simulink model "test_2_SPI"  (Simulink 7.1)
settings: Solver=FixedStepDiscrete  StartTime=0.0  StopTime=10.0  FixedStep=0.001  RelTol=1e-3
libraries: dsPICdrivers x4
settings Model: Creator=Huysman Michael  LastModifiedBy=Huysman Michael
settings OptimizationCC: OptimizeModelRefInitCode=on  LifeSpan=1
settings HardwareCC: ProdBitPerInt=16  ProdEndianess=LittleEndian  ProdWordSize=16  ProdHWDeviceType=16-bit Generic
settings RTWCC: SystemTargetFile=dspic.tlc  TemplateMakefile=dspic_pic30_gcc.tmf  PostCodeGenCommand=dsPIC_Compile()  Description=Embedded Target for Microchip dsPIC (real-time)  ProcessScript=dspic_make_rtw_hook
settings CodeAppCC: IgnoreCustomStorageClasses=off
settings STFCustomTargetCC: ModelReferenceCompliant=off  IncludeMdlTerminateFcn=off  CombineOutputUpdateFcns=on  SuppressErrorStatus=on  ERTCustomFileBanners=on  SupportContinuousTime=off  SupportNonInlinedSFcns=off  SystemTargetFile=dspic.tlc
settings ERTTargetCC: ModelReferenceCompliant=off  CompOptLevelCompliant=off  IncludeMdlTerminateFcn=off  SuppressErrorStatus=on  ERTFirstTimeCompliant=off  ModelStepFunctionPrototypeControlCompliant=off  ExtModeMexFile=noextcomm  InlinedParameterPlacement=NonHierarchical  ERTSrcFileBannerTemplate=dsPIC_code_template.cgt  ERTHdrFileBannerTemplate=dsPIC_code_template.cgt  ERTDataSrcFileTemplate=dsPIC_code_template.cgt  ERTDataHdrFileTemplate=dsPIC_code_template.cgt  ERTCustomFileTemplate=dsPIC_main.tlc
settings CustomProperty: DataType=string  Value=C:\PROGRA~1\MATLAB~1\R2008a\bin\win32\gmake

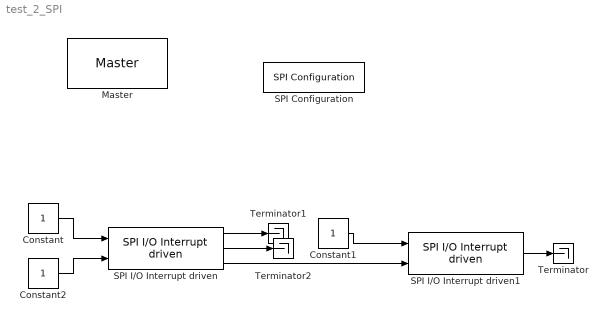
== system test_2_SPI ==
  Constant : Constant  OutDataTypeMode=uint16  OutDataType=sfix(16)  OutScaling=2^0  OutDataTypeStr=uint16
  Constant1 : Constant  OutDataTypeMode=uint16  OutDataType=sfix(16)  OutScaling=2^0  OutDataTypeStr=uint16
  Constant2 : Constant  OutDataTypeMode=uint16  OutDataType=sfix(16)  OutScaling=2^0  OutDataTypeStr=uint16
  Master : dsPICdrivers/Master  Tag=dsPIC_MASTER  Priority=1  TimeStepType=Timer1  picType=33fJ256GP710  fcy=2500000  Quartz_33f=5e6  PLLActive_33f=off  fcyDesired_33f=0  tmr1="[1  2499  0]"  tmr1Info="Time Step : 0.001  ;   Error : 0%  PR1=2499"  tmr2345="[0  0  0  0  0  0  0  0]"  tmr2345cfg=[-1 -1 -1 -1 -1 -1 -1 -1]  IOautoConf=on  typePort="[ 0   0   0   0   0   0   0   0   0   0   0   0   0   0   0   0   0   0   0   0   0   0   0   0   0   0   0   0   0   0   0   0   0   0   0   0   0   0   0   0   0   0   0   0   0   0   0   0   0   0   0   0   0   0   0   0   0   0   0   0   0   0   0   0   0   0   0   0   0   0   0   0   0   0   0   0   0   0   0   0   0   0   0   0   0   0  17   0   0   0   0   0   0   0   0   0   0   0   0   0   0   0   0   0   0   0   0   0   0   0   0   0 ]"  TRIS="[ 65535  65535  65535  65535  65535  65535  65535 ]"  ADPCFG=0  MasterBusyPort=None  MasterOverloadPort=None  FOSC=Quartz (XT - HS)  TempProtection_33f=TEMP_ON  FPBOR=<empty>  PWRT=disable  MCLR=<empty>  PowerSave=off
  SPI Configuration : dsPICdrivers/SPI PORT/SPI Configuration  Tag=dsPIC_config_SPI  Priority=2  ConfigurationTime=At boot time (only once)  OrderingInOutPopup=None  SampleTime=-1  Frame_Enable=0  Frame_Sync=None  SPI=1  MODE=MASTER  USER_SCALER=20  StartEnable=Enable  SDO_EN=off  DATA_LENGTH=16 bits  SS_EN=off  SMP=End of bit  CKP=high  CKE=Idle to Active  Status="OK - Mode 1  -    Fsck= 125000Hz"
  SPI I/O Interrupt driven : dsPICdrivers/SPI PORT/SPI I//O Interrupt driven  Tag=dsPIC_SPI_IO_Interrupt  SPI=1  nbrTrame=2  mode=continuous run - interrupt disable after block execution (need reenable)  Disable=off  DATA_LENGTH=16 bits  OrderingInOutPopup=Output  SampleTime=-1  T1CSL=None  T1CSH=None  T2CSL=None  T2CSH=None  T3CSL=None  T3CSH=None  T4CSL=None  T4CSH=None  T5CSL=None  T5CSH=None  T6CSL=None  T6CSH=None  T7CSL=None  T7CSH=None  T8CSL=None  T8CSH=None  T9CSL=None  T9CSH=None  T10CSL=None  T10CSH=None  T11CSL=None  T11CSH=None  T12CSL=None  T12CSH=None  T13CSL=None  T13CSH=None  T14CSL=None  T14CSH=None  T15CSL=None  T15CSH=None
  SPI I/O Interrupt driven1 : dsPICdrivers/SPI PORT/SPI I//O Interrupt driven  Tag=dsPIC_SPI_IO_Interrupt  SPI=1  nbrTrame=1  mode=continuous run - interrupt disable after block execution (need reenable)  Disable=off  DATA_LENGTH=16 bits  OrderingInOutPopup=Input  SampleTime=-1  T1CSL=None  T1CSH=None  T2CSL=None  T2CSH=None  T3CSL=None  T3CSH=None  T4CSL=None  T4CSH=None  T5CSL=None  T5CSH=None  T6CSL=None  T6CSH=None  T7CSL=None  T7CSH=None  T8CSL=None  T8CSH=None  T9CSL=None  T9CSH=None  T10CSL=None  T10CSH=None  T11CSL=None  T11CSH=None  T12CSL=None  T12CSH=None  T13CSL=None  T13CSH=None  T14CSL=None  T14CSH=None  T15CSL=None  T15CSH=None
  Terminator : Terminator
  Terminator1 : Terminator
  Terminator2 : Terminator
  wires:
  Constant1/1 -> SPI I/O Interrupt driven1/1
  Constant/1 -> SPI I/O Interrupt driven/1
  SPI I/O Interrupt driven1/1 -> Terminator/1
  Constant2/1 -> SPI I/O Interrupt driven/2
  SPI I/O Interrupt driven/3 -> SPI I/O Interrupt driven1/2
  SPI I/O Interrupt driven/1 -> Terminator1/1
  SPI I/O Interrupt driven/2 -> Terminator2/1
